simulink model "Standalone_AnalogGeneration"  (R2024b)
settings: Solver=FixedStepAuto  StartTime=0.0  StopTime=inf  RelTol=1e-3
undefined symbols (not defined in the file): IO397, pull, up
libraries: speedgoatlib_fpga_analog_io x1, speedgoatlib_fpga x1
settings Model: SimulationMode=external  Creator=rodri  LastModifiedBy=rodri
settings SolverCC: ConcurrentTasks=on  PositivePriorityOrder=on
settings OptimizationCC: BlockReduction=off  OptimizeBlockIOStorage=off
settings DebuggingCC: TasksWithSamePriorityMsg=none
settings HardwareCC: ProdBitPerLong=64  ProdLongLongMode=on  ProdHWDeviceType=Intel->x86-64 (Linux 64)
settings RTWCC: Description=Speedgoat Real-Time Target Machine  SystemTargetFile=speedgoat.tlc  TemplateMakefile=slrealtime_default_tmf  Toolchain=Simulink Real-Time Toolchain  BuildConfiguration=Faster Runs  CodeExecutionProfiling=on  TargetLang=C++  GPUComputeCapability=3.5
settings SimulinkRealTimeTargetCC: InstructionSetFMA=off  LogToMDFFile=off

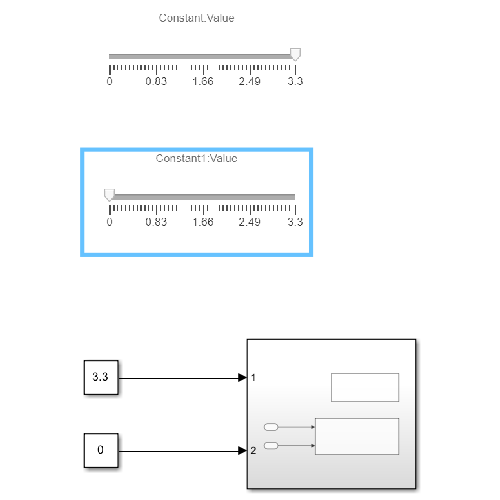
[thumbnail: Simulink's stored preview of the top-level diagram]
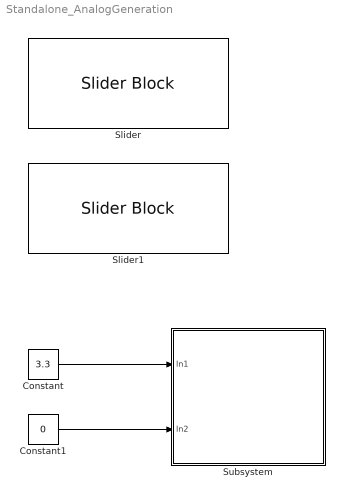
== system Standalone_AnalogGeneration ==
  Constant : Constant  Value=3.3  OutMin=0  OutMax=3.3  SampleTime=-1
  Constant1 : Constant  Value=0  OutMin=0  OutMax=3.3  SampleTime=-1
  Slider : SliderBlock  ScaleMax=3.3
  Slider1 : SliderBlock  ScaleMax=3.3
  Subsystem : Subsystem
  wires:
  Constant/1 -> Subsystem/1(In1)
  Constant1/1 -> Subsystem/2(In2)

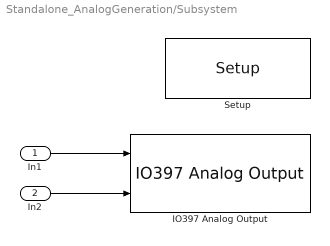
== system Standalone_AnalogGeneration/Subsystem ==
  In1 : Inport
  In2 : Inport  Port=2
  IO397 Analog Output : speedgoatlib_fpga_analog_io/IO397/IO397 Analog Output  id=1  chan=[1 2]  initVal=0  resetVal=0  ts=0.001  span=+5 V
      settings: SourceProductName=Analog IO
  Setup : speedgoatlib_fpga/Setup/Setup  Parameter124={}  board=IO397-50k  id=1  pciSlot=-1  device_id=1  bitstreamFilePath=C:\ProgramData\Speedgoat\bitstreams\io_configuration_package\R2024b\io397  bitstreamFile=speedgoat_IO397_HIL.mat  rearEnb_1=off  rearIO_1=None  rearEnb_2=off  rearIO_2=None  ProgSpiFlash=off  ProgBPIFlash=off  useFpgaDmaController=off  PullRPort15=pull-up 3.3V  PullRPort31=pull-up 3.3V  PullRPort47=pull-up 3.3V  PullRPort63=pull-up 3.3V  diffLineTermination_1=on  diffLineTermination_2=on  diffLineTermination_3=on  diffLineTermination_4=on  diffLineTermination_5=on  diffLineTermination_6=on  diffLineTermination_7=on  diffLineTermination_8=on  diffLineTermination_9=on  diffLineTermination_10=on  diffLineTermination_11=on  diffLineTermination_12=on  diffLineTermination_13=on  diffLineTermination_14=on  diffLineTermination_15=on  diffLineTermination_16=on  diffLineTermination_17=on  diffLineTermination_18=on  diffLineTermination_19=on  diffLineTermination_20=on  diffLineTermination_21=on  diffLineTermination_22=on  diffLineTermination_23=on  diffLineTermination_24=on  diffLineTermination_25=on  diffLineTermination_26=on  diffLineTermination_27=on  diffLineTermination_28=on  diffLineTermination_29=on  diffLineTermination_30=on  diffLineTermination_31=on  diffLineTermination_32=on  Vi_Pull_36x_1=Floating  Vo_36x_1=3.3V  Vi_Pull_36x_2=Floating  Vo_36x_2=3.3V  Vi_Pull_36x_3=Floating  Vo_36x_3=3.3V  Vi_Pull_36x_4=Floating  Vo_36x_4=3.3V  Vi_Pull_36x_5=Floating  Vo_36x_5=3.3V  Vi_Pull_36x_6=Floating  Vo_36x_6=3.3V  Vi_Pull_36x_7=Floating  Vo_36x_7=3.3V  Vi_Pull_36x_8=Floating  Vo_36x_8=3.3V  Vi_Pull_36x_9_16=Floating  Vo_36x_9_16=3.3V  Vi_Pull_36x_17_24=Floating  Vo_36x_17_24=3.3V  Vi_Pull_36x_25_32=Floating  Vo_36x_25_32=3.3V  Vi_Pull_36x_33_40=Floating  Vo_36x_33_40=3.3V  Vi_Pull_36x_41_48=Floating  Vo_36x_41_48=3.3V  Vi_Pull_36x_49_56=Floating  Vo_36x_49_56=3.3V  Vi_Pull_36x_57_64=Floating  Vo_36x_57_64=3.3V  PullRPort0_1=pull-up  VioPort0_1=3.3V  PullRPort1_1=pull-up  VioPort1_1=3.3V  PullRPort2_1=pull-up  VioPort2_1=3.3V  PullRPort3_1=pull-up  VioPort3_1=3.3V  PullRPort4_1=pull-up  VioPort4_1=3.3V  PullRPort5_1=pull-up  VioPort5_1=3.3V  PullRPort6_1=pull-up  VioPort6_1=3.3V  diffLineTermination_rear1_1=on  diffLineTermination_rear1_2=on  diffLineTermination_rear1_3=on  diffLineTermination_rear1_4=on  diffLineTermination_rear1_5=on  diffLineTermination_rear1_6=on  diffLineTermination_rear1_7=on  diffLineTermination_rear1_8=on  PullRPort0_2=pull-up  VioPort0_2=3.3V  PullRPort1_2=pull-up  VioPort1_2=3.3V  PullRPort2_2=pull-up  VioPort2_2=3.3V  PullRPort3_2=pull-up  VioPort3_2=3.3V  PullRPort4_2=pull-up  VioPort4_2=3.3V  PullRPort5_2=pull-up  VioPort5_2=3.3V  PullRPort6_2=pull-up  VioPort6_2=3.3V  diffLineTermination_rear2_1=on  diffLineTermination_rear2_2=on  diffLineTermination_rear2_3=on  diffLineTermination_rear2_4=on  diffLineTermination_rear2_5=on  diffLineTermination_rear2_6=on  diffLineTermination_rear2_7=on  diffLineTermination_rear2_8=on
      settings: SourceProductName=IO3xx
  wires:
  In2/1 -> IO397 Analog Output/2
  In1/1 -> IO397 Analog Output/1
